simulink model "sm_car"  (R2025a)
settings: Solver=ode23t  StartTime=0.0  StopTime=400  MaxStep=0.4  RelTol=1e-3  AbsTol=1e-3  EnableMultiTasking=on
PreLoadFcn:
  | % Due to usability issue in Repeating Sequence block
  | warning('off','Simulink:Masking:Invalid');
  | 
  | % Eliminate unnecessary warnings in inactive variants
  | % Warnings generated only if you click through inactive variant
  | warning('off','MATLAB:nonExistentField');
  | warning('off','Simulink:Parameters:BlkParamUndefined');
PostLoadFcn:
  | set_param([bdroot '/Vehicle'],'popup_trailer','Off')
  | warning('off','sm:sli:setup:compile:LocalSolverNotSupported')
  | %sm_car_config_maneuver(bdroot,'WOT Braking');
  | sm_car_config_vehicle(bdroot,'false');
  | sm_car_config_logging(bdroot);
InitFcn:
  | sm_car_config_camera;
  | Vehicle = sm_car_vehcfg_checkConfig(Vehicle);
  | sm_car_check_tire_model(bdroot);
StartFcn:
  | tic;
StopFcn:
  | Elapsed_Sim_Time = toc;
  | % disp(['Elapsed Sim Time = ' num2str(Elapsed_Sim_Time)]);
undefined symbols (not defined in the file): Axle1D, AxleIn, Camera, Control, Driver, Free, Init, Maneuver, Pedal, RaceFix, RaceSpin, Scene, ShaftL1, ShaftL2, ShaftR1, ShaftR2, Soft, Stiff, Visual, X, xy_data_car_side, Y, Z
libraries: sm_lib x1546, nesl_utility x528, fl_lib x480, SimscapeFluids_lib x61, sdl_lib x49, simulink x29, ee_lib x7, simulink_extras x6, Linkage_Systems x4, Tire_1x2x x4, AntiRollBar_Systems x2, Linkage_Decoupled x2
(part 22 of 79)

== system sm_car/Vehicle/Vehicle/Chassis/Body/Body Geometry/CAD FSAE Achilles/Aero ==
  Aero Brackets : sm_lib/Body Elements/File Solid  ExtGeomFileName=FSAE_Aero_Brackets.STL  UnitType=Custom  ExtGeomFileUnits=m  StepReaderType=HEX  ExportConvexHullGeometry=off  InertiaType=PointMass  BasedOnType=Density  Density=700.769  DensityUnits=kg/m^3  Mass=0  MassUnits=kg  CenterOfMass=[0.988684, 1.00464/1.8, 2.92072]  CenterOfMassUnits=m  MomentsOfInertia=[478.463, 518.088, 108.52]  MomentsOfInertiaUnits=kg*m^2  ProductsOfInertia=[-18.6469, 0.0347848, 0.00267861]  ProductsOfInertiaUnits=kg*m^2  GraphicType=FromGeometry  MarkerShape=Sphere  MarkerSize=10  GraphicVisPropType=SimpleVisualProperties  GraphicDiffuseColor=[0.25 0.25 0.25]  GraphicOpacity=1  GraphicSpecularColor=[0.5 0.5 0.5 1.0]  GraphicAmbientColor=[0.15 0.15 0.15 1.0]  GraphicEmissiveColor=[0.0 0.0 0.0 1.0]  GraphicShininess=75  DoExposeReferenceFrame=on  SerializedFrames=<Frames/>
  Aero Surfaces : sm_lib/Body Elements/File Solid  ExtGeomFileName=FSAE_Aero_Surfaces.STL  UnitType=Custom  ExtGeomFileUnits=m  StepReaderType=HEX  ExportConvexHullGeometry=off  InertiaType=PointMass  BasedOnType=Density  Density=700.769  DensityUnits=kg/m^3  Mass=0  MassUnits=kg  CenterOfMass=[0.988684, 1.00464/1.8, 2.92072]  CenterOfMassUnits=m  MomentsOfInertia=[478.463, 518.088, 108.52]  MomentsOfInertiaUnits=kg*m^2  ProductsOfInertia=[-18.6469, 0.0347848, 0.00267861]  ProductsOfInertiaUnits=kg*m^2  GraphicType=FromGeometry  MarkerShape=Sphere  MarkerSize=10  GraphicVisPropType=SimpleVisualProperties  GraphicDiffuseColor=aero_clr  GraphicOpacity=aero_opc  GraphicSpecularColor=[0.5 0.5 0.5 1.0]  GraphicAmbientColor=[0.15 0.15 0.15 1.0]  GraphicEmissiveColor=[0.0 0.0 0.0 1.0]  GraphicShininess=75  DoExposeReferenceFrame=on  SerializedFrames=<Frames/>
  Ornament Left : sm_lib/Body Elements/Extruded Solid  ExtrusionType=General  PolygonNumSides=3  PolygonOuterRadius=1  PolygonOuterRadiusUnits=m  ExportEntireGeometry=off  ExtrusionCrossSection=extr_data_emblem_aero  ExtrusionCrossSectionUnits=m  ExportConvexHullGeometry=off  ExtrusionLength=0.005  ExtrusionLengthUnits=m  InertiaType=CalculateFromGeometry  BasedOnType=Density  Density=1000  DensityUnits=kg/m^3  Mass=1  MassUnits=kg  CenterOfMass=[0 0 0]  CenterOfMassUnits=m  MomentsOfInertia=[1 1 1]  MomentsOfInertiaUnits=kg*m^2  ProductsOfInertia=[0 0 0]  ProductsOfInertiaUnits=kg*m^2  GraphicType=FromGeometry  MarkerShape=Sphere  MarkerSize=10  GraphicVisPropType=SimpleVisualProperties  GraphicDiffuseColor=clr_emblem_aero  GraphicOpacity=opc_emblem_aero  GraphicSpecularColor=[0.5 0.5 0.5 1.0]  GraphicAmbientColor=[0.15 0.15 0.15 1.0]  GraphicEmissiveColor=[0.0 0.0 0.0 1.0]  GraphicShininess=75  DoExposeReferenceFrame=on  SerializedFrames=<Frames/>
  Ornament Right : sm_lib/Body Elements/Extruded Solid  ExtrusionType=General  PolygonNumSides=3  PolygonOuterRadius=1  PolygonOuterRadiusUnits=m  ExportEntireGeometry=off  ExtrusionCrossSection=extr_data_emblem_aero  ExtrusionCrossSectionUnits=m  ExportConvexHullGeometry=off  ExtrusionLength=0.005  ExtrusionLengthUnits=m  InertiaType=CalculateFromGeometry  BasedOnType=Density  Density=1000  DensityUnits=kg/m^3  Mass=1  MassUnits=kg  CenterOfMass=[0 0 0]  CenterOfMassUnits=m  MomentsOfInertia=[1 1 1]  MomentsOfInertiaUnits=kg*m^2  ProductsOfInertia=[0 0 0]  ProductsOfInertiaUnits=kg*m^2  GraphicType=FromGeometry  MarkerShape=Sphere  MarkerSize=10  GraphicVisPropType=SimpleVisualProperties  GraphicDiffuseColor=clr_emblem_aero  GraphicOpacity=opc_emblem_aero  GraphicSpecularColor=[0.5 0.5 0.5 1.0]  GraphicAmbientColor=[0.15 0.15 0.15 1.0]  GraphicEmissiveColor=[0.0 0.0 0.0 1.0]  GraphicShininess=75  DoExposeReferenceFrame=on  SerializedFrames=<Frames/>
  Transform Aero Ctr : sm_lib/Frames and Transforms/Rigid Transform  RotationMethod=None  FollAlignAxisA=+X  BaseAlignAxisA=+Y  FollAlignAxisB=+Y  BaseAlignAxisB=+Z  RotationStandardAxis=+X  RotationAngle=90  RotationAngleUnits=deg  RotationArbitraryAxis=[0 0 1]  RotationSequenceAxes=FollowerAxes  RotationSequence=XYX  RotationSequenceAngles=[0 0 0]  RotationSequenceAnglesUnits=deg  RotationMatrix=[1 0 0;0 1 0;0 0 1]  Quaternion=[1 0 0 0]  TranslationMethod=Cartesian  TranslationCartesianOffset=[-1.15 0 0.75]  TranslationCartesianOffsetUnits=m  TranslationStandardAxis=+Z  TranslationStandardOffset=0  TranslationStandardOffsetUnits=m  TranslationROffset=0  TranslationROffsetUnits=m  TranslationThetaOffset=0  TranslationThetaOffsetUnits=deg  TranslationZOffset=0  TranslationZOffsetUnits=m
  Transform Aero Left : sm_lib/Frames and Transforms/Rigid Transform  RotationMethod=RotationSequence  FollAlignAxisA=+X  BaseAlignAxisA=+Y  FollAlignAxisB=+Y  BaseAlignAxisB=+Z  RotationStandardAxis=+X  RotationAngle=90  RotationAngleUnits=deg  RotationArbitraryAxis=[0 0 1]  RotationSequenceAxes=FollowerAxes  RotationSequence=XYX  RotationSequenceAngles=[90 180 0]  RotationSequenceAnglesUnits=deg  RotationMatrix=[1 0 0;0 1 0;0 0 1]  Quaternion=[1 0 0 0]  TranslationMethod=Cartesian  TranslationCartesianOffset=[0 0.465 0]  TranslationCartesianOffsetUnits=m  TranslationStandardAxis=+Z  TranslationStandardOffset=0  TranslationStandardOffsetUnits=m  TranslationROffset=0  TranslationROffsetUnits=m  TranslationThetaOffset=0  TranslationThetaOffsetUnits=deg  TranslationZOffset=0  TranslationZOffsetUnits=m
  Transform Aero Right : sm_lib/Frames and Transforms/Rigid Transform  RotationMethod=StandardAxis  FollAlignAxisA=+X  BaseAlignAxisA=+Y  FollAlignAxisB=+Y  BaseAlignAxisB=+Z  RotationStandardAxis=+X  RotationAngle=90  RotationAngleUnits=deg  RotationArbitraryAxis=[0 0 1]  RotationSequenceAxes=FollowerAxes  RotationSequence=XYX  RotationSequenceAngles=[0 0 0]  RotationSequenceAnglesUnits=deg  RotationMatrix=[1 0 0;0 1 0;0 0 1]  Quaternion=[1 0 0 0]  TranslationMethod=Cartesian  TranslationCartesianOffset=[0 -0.465 0]  TranslationCartesianOffsetUnits=m  TranslationStandardAxis=+Z  TranslationStandardOffset=0  TranslationStandardOffsetUnits=m  TranslationROffset=0  TranslationROffsetUnits=m  TranslationThetaOffset=0  TranslationThetaOffsetUnits=deg  TranslationZOffset=0  TranslationZOffsetUnits=m
  R : PMIOPort  Side=Right
  connections:
  Ornament Right/RConn1 -- Transform Aero Right/RConn1
  Ornament Left/RConn1 -- Transform Aero Left/RConn1
  Aero Surfaces/RConn1 -- Transform Aero Ctr/LConn1 -- R/RConn1 -- Aero Brackets/RConn1
  Transform Aero Ctr/RConn1 -- Transform Aero Left/LConn1 -- Transform Aero Right/LConn1

== system sm_car/Vehicle/Vehicle/Chassis/Body/Body Geometry/CAD FSAE Achilles/Body ==
  Ornament Hood : sm_lib/Body Elements/Extruded Solid  ExtrusionType=General  PolygonNumSides=3  PolygonOuterRadius=1  PolygonOuterRadiusUnits=m  ExportEntireGeometry=off  ExtrusionCrossSection=extr_data_emblem_hood  ExtrusionCrossSectionUnits=m  ExportConvexHullGeometry=off  ExtrusionLength=0.01  ExtrusionLengthUnits=m  InertiaType=CalculateFromGeometry  BasedOnType=Density  Density=1000  DensityUnits=kg/m^3  Mass=1  MassUnits=kg  CenterOfMass=[0 0 0]  CenterOfMassUnits=m  MomentsOfInertia=[1 1 1]  MomentsOfInertiaUnits=kg*m^2  ProductsOfInertia=[0 0 0]  ProductsOfInertiaUnits=kg*m^2  GraphicType=FromGeometry  MarkerShape=Sphere  MarkerSize=10  GraphicVisPropType=SimpleVisualProperties  GraphicDiffuseColor=clr_emblem_hood  GraphicOpacity=opc_emblem_hood  GraphicSpecularColor=[0.5 0.5 0.5 1.0]  GraphicAmbientColor=[0.15 0.15 0.15 1.0]  GraphicEmissiveColor=[0.0 0.0 0.0 1.0]  GraphicShininess=75  DoExposeReferenceFrame=on  SerializedFrames=<Frames/>
  Shell : sm_lib/Body Elements/File Solid  ExtGeomFileName=FSAE_Body.STL  UnitType=Custom  ExtGeomFileUnits=m  StepReaderType=HEX  ExportConvexHullGeometry=off  InertiaType=PointMass  BasedOnType=Density  Density=700.769  DensityUnits=kg/m^3  Mass=0  MassUnits=kg  CenterOfMass=[0.988684, 1.00464/1.8, 2.92072]  CenterOfMassUnits=m  MomentsOfInertia=[478.463, 518.088, 108.52]  MomentsOfInertiaUnits=kg*m^2  ProductsOfInertia=[-18.6469, 0.0347848, 0.00267861]  ProductsOfInertiaUnits=kg*m^2  GraphicType=FromGeometry  MarkerShape=Sphere  MarkerSize=10  GraphicVisPropType=SimpleVisualProperties  GraphicDiffuseColor=[body_clr]  GraphicOpacity=body_opc  GraphicSpecularColor=[0.5 0.5 0.5 body_opc]  GraphicAmbientColor=[body_clr body_opc]  GraphicEmissiveColor=[0.0 0.0 0.0 body_opc]  GraphicShininess=50  DoExposeReferenceFrame=on  SerializedFrames=<Frames/>
  Transform Hood : sm_lib/Frames and Transforms/Rigid Transform  RotationMethod=RotationSequence  FollAlignAxisA=+X  BaseAlignAxisA=+Y  FollAlignAxisB=+Y  BaseAlignAxisB=+Z  RotationStandardAxis=+X  RotationAngle=90  RotationAngleUnits=deg  RotationArbitraryAxis=[0 0 1]  RotationSequenceAxes=FollowerAxes  RotationSequence=ZXY  RotationSequenceAngles=[90 9 0]  RotationSequenceAnglesUnits=deg  RotationMatrix=[1 0 0;0 1 0;0 0 1]  Quaternion=[1 0 0 0]  TranslationMethod=Cartesian  TranslationCartesianOffset=[0.75 0 0.56]  TranslationCartesianOffsetUnits=m  TranslationStandardAxis=+Z  TranslationStandardOffset=0  TranslationStandardOffsetUnits=m  TranslationROffset=0  TranslationROffsetUnits=m  TranslationThetaOffset=0  TranslationThetaOffsetUnits=deg  TranslationZOffset=0  TranslationZOffsetUnits=m
  R : PMIOPort  Side=Left
  connections:
  Shell/RConn1 -- R/RConn1 -- Transform Hood/LConn1
  Transform Hood/RConn1 -- Ornament Hood/RConn1

== system sm_car/Vehicle/Vehicle/Chassis/Body/Body Sensor/Roll Pitch/Calculate aPitch ==
  Roll Angle : Inport
  uvec : Inport  Port=2
  Asin : Trigonometry  Operator=asin
  Cos : Trigonometry  Operator=cos
  Divide : Product  Inputs=*/
  Divide1 : Product  Inputs=*/
  Selector : Selector  InputPortWidth=3  IndexOptions=Index vector (dialog)  Indices=[3]  OutputSizes=1
  magnitude : Fcn  Expr=sqrt(u(1)*u(1)+u(2)*u(2)+u(3)*u(3))
  Angle : Outport  VectorParamsAs1DForOutWhenUnconnected=off
  wires:
  Divide1/1 -> Asin/1
  uvec/1 -> magnitude/1, Selector/1
  magnitude/1 -> Divide1/2
  Selector/1 -> Divide/1
  Roll Angle/1 -> Cos/1
  Asin/1 -> Angle/1
  Divide/1 -> Divide1/1
  Cos/1 -> Divide/2

== system sm_car/Vehicle/Vehicle/Chassis/Body/Body Sensor/Roll Pitch/Calculate aRoll ==
  uvec : Inport
  Demux : Demux  Outputs=3
  Mux : Mux  Inputs=2
  Trigonometric Function1 : Trigonometry  Operator=atan2
  magnitude : Fcn  Expr=sqrt(u(1)*u(1)+u(2)*u(2))
  Angle : Outport  VectorParamsAs1DForOutWhenUnconnected=off
  wires:
  Demux/2 -> Mux/2
  magnitude/1 -> Trigonometric Function1/2
  Mux/1 -> magnitude/1
  Demux/3 -> Trigonometric Function1/1
  Trigonometric Function1/1 -> Angle/1
  uvec/1 -> Demux/1
  Demux/1 -> Mux/1

== system sm_car/Vehicle/Vehicle/Chassis/Body/Passenger FL/None/Body Sensor Empty ==
  Constant{,1..14} (15 alike) : Constant  Value=0
  Reference Frame : sm_lib/Frames and Transforms/Reference Frame
  Signal Specification : SignalSpecification  Unit=rad
  Signal Specification1 : SignalSpecification  Unit=rad
  Signal Specification2 : SignalSpecification  Unit=rad
  Signal Specification3 : SignalSpecification  Unit=rad/s
  Signal Specification4 : SignalSpecification  Unit=rad/s
  Signal Specification5 : SignalSpecification  Unit=rad/s
  B : PMIOPort  Side=Left
  Bus Element Out : Outport  VectorParamsAs1DForOutWhenUnconnected=off  PortName=Body  Element=x
  Bus Element Out1 : Outport  VectorParamsAs1DForOutWhenUnconnected=off  PortName=Body  Element=y
  Bus Element Out2 : Outport  VectorParamsAs1DForOutWhenUnconnected=off  PortName=Body  Element=z
  Bus Element Out3 : Outport  VectorParamsAs1DForOutWhenUnconnected=off  PortName=Body  Element=vx
  Bus Element Out4 : Outport  VectorParamsAs1DForOutWhenUnconnected=off  PortName=Body  Element=vy
  Bus Element Out5 : Outport  VectorParamsAs1DForOutWhenUnconnected=off  PortName=Body  Element=vz
  Bus Element Out6 : Outport  VectorParamsAs1DForOutWhenUnconnected=off  PortName=Body  Element=gx
  Bus Element Out7 : Outport  VectorParamsAs1DForOutWhenUnconnected=off  PortName=Body  Element=gy
  Bus Element Out8 : Outport  VectorParamsAs1DForOutWhenUnconnected=off  PortName=Body  Element=gz
  Bus Element Out9 : Outport  VectorParamsAs1DForOutWhenUnconnected=off  PortName=Body  Element=nRoll
  Bus Element Out10 : Outport  VectorParamsAs1DForOutWhenUnconnected=off  PortName=Body  Element=nPitch
  Bus Element Out11 : Outport  VectorParamsAs1DForOutWhenUnconnected=off  PortName=Body  Element=nYaw
  Bus Element Out12 : Outport  VectorParamsAs1DForOutWhenUnconnected=off  PortName=Body  Element=aRoll
  Bus Element Out13 : Outport  VectorParamsAs1DForOutWhenUnconnected=off  PortName=Body  Element=aPitch
  Bus Element Out14 : Outport  VectorParamsAs1DForOutWhenUnconnected=off  PortName=Body  Element=aYaw
  wires:
  Constant2/1 -> Signal Specification/1
  Constant3/1 -> Signal Specification1/1
  Constant5/1 -> Signal Specification4/1
  Constant4/1 -> Signal Specification3/1
  Constant1/1 -> Signal Specification5/1
  Constant/1 -> Signal Specification2/1
  Signal Specification5/1 -> Bus Element Out11/1
  Signal Specification4/1 -> Bus Element Out10/1
  Signal Specification3/1 -> Bus Element Out9/1
  Signal Specification2/1 -> Bus Element Out14/1
  Signal Specification1/1 -> Bus Element Out13/1
  Signal Specification/1 -> Bus Element Out12/1
  Constant9/1 -> Bus Element Out3/1
  Constant6/1 -> Bus Element Out/1
  Constant8/1 -> Bus Element Out2/1
  Constant10/1 -> Bus Element Out4/1
  Constant13/1 -> Bus Element Out7/1
  Constant7/1 -> Bus Element Out1/1
  Constant12/1 -> Bus Element Out6/1
  Constant11/1 -> Bus Element Out5/1
  Constant14/1 -> Bus Element Out8/1
  connections:
  B/RConn1 -- Reference Frame/RConn1

== system sm_car/Vehicle/Vehicle/Chassis/Body/Passenger FR/None/Body Sensor Empty ==
  Constant{,1..14} (15 alike) : Constant  Value=0
  Reference Frame : sm_lib/Frames and Transforms/Reference Frame
  Signal Specification : SignalSpecification  Unit=rad
  Signal Specification1 : SignalSpecification  Unit=rad
  Signal Specification2 : SignalSpecification  Unit=rad
  Signal Specification3 : SignalSpecification  Unit=rad/s
  Signal Specification4 : SignalSpecification  Unit=rad/s
  Signal Specification5 : SignalSpecification  Unit=rad/s
  B : PMIOPort  Side=Left
  Bus Element Out : Outport  VectorParamsAs1DForOutWhenUnconnected=off  PortName=Body  Element=x
  Bus Element Out1 : Outport  VectorParamsAs1DForOutWhenUnconnected=off  PortName=Body  Element=y
  Bus Element Out2 : Outport  VectorParamsAs1DForOutWhenUnconnected=off  PortName=Body  Element=z
  Bus Element Out3 : Outport  VectorParamsAs1DForOutWhenUnconnected=off  PortName=Body  Element=vx
  Bus Element Out4 : Outport  VectorParamsAs1DForOutWhenUnconnected=off  PortName=Body  Element=vy
  Bus Element Out5 : Outport  VectorParamsAs1DForOutWhenUnconnected=off  PortName=Body  Element=vz
  Bus Element Out6 : Outport  VectorParamsAs1DForOutWhenUnconnected=off  PortName=Body  Element=gx
  Bus Element Out7 : Outport  VectorParamsAs1DForOutWhenUnconnected=off  PortName=Body  Element=gy
  Bus Element Out8 : Outport  VectorParamsAs1DForOutWhenUnconnected=off  PortName=Body  Element=gz
  Bus Element Out9 : Outport  VectorParamsAs1DForOutWhenUnconnected=off  PortName=Body  Element=nRoll
  Bus Element Out10 : Outport  VectorParamsAs1DForOutWhenUnconnected=off  PortName=Body  Element=nPitch
  Bus Element Out11 : Outport  VectorParamsAs1DForOutWhenUnconnected=off  PortName=Body  Element=nYaw
  Bus Element Out12 : Outport  VectorParamsAs1DForOutWhenUnconnected=off  PortName=Body  Element=aRoll
  Bus Element Out13 : Outport  VectorParamsAs1DForOutWhenUnconnected=off  PortName=Body  Element=aPitch
  Bus Element Out14 : Outport  VectorParamsAs1DForOutWhenUnconnected=off  PortName=Body  Element=aYaw
  wires:
  Constant2/1 -> Signal Specification/1
  Constant3/1 -> Signal Specification1/1
  Constant5/1 -> Signal Specification4/1
  Constant4/1 -> Signal Specification3/1
  Constant1/1 -> Signal Specification5/1
  Constant/1 -> Signal Specification2/1
  Signal Specification5/1 -> Bus Element Out11/1
  Signal Specification4/1 -> Bus Element Out10/1
  Signal Specification3/1 -> Bus Element Out9/1
  Signal Specification2/1 -> Bus Element Out14/1
  Signal Specification1/1 -> Bus Element Out13/1
  Signal Specification/1 -> Bus Element Out12/1
  Constant9/1 -> Bus Element Out3/1
  Constant6/1 -> Bus Element Out/1
  Constant8/1 -> Bus Element Out2/1
  Constant10/1 -> Bus Element Out4/1
  Constant13/1 -> Bus Element Out7/1
  Constant7/1 -> Bus Element Out1/1
  Constant12/1 -> Bus Element Out6/1
  Constant11/1 -> Bus Element Out5/1
  Constant14/1 -> Bus Element Out8/1
  connections:
  B/RConn1 -- Reference Frame/RConn1

== system sm_car/Vehicle/Vehicle/Chassis/Body/Passenger RL/None/Body Sensor Empty ==
  Constant{,1..14} (15 alike) : Constant  Value=0
  Reference Frame : sm_lib/Frames and Transforms/Reference Frame
  Signal Specification : SignalSpecification  Unit=rad
  Signal Specification1 : SignalSpecification  Unit=rad
  Signal Specification2 : SignalSpecification  Unit=rad
  Signal Specification3 : SignalSpecification  Unit=rad/s
  Signal Specification4 : SignalSpecification  Unit=rad/s
  Signal Specification5 : SignalSpecification  Unit=rad/s
  B : PMIOPort  Side=Left
  Bus Element Out : Outport  VectorParamsAs1DForOutWhenUnconnected=off  PortName=Body  Element=x
  Bus Element Out1 : Outport  VectorParamsAs1DForOutWhenUnconnected=off  PortName=Body  Element=y
  Bus Element Out2 : Outport  VectorParamsAs1DForOutWhenUnconnected=off  PortName=Body  Element=z
  Bus Element Out3 : Outport  VectorParamsAs1DForOutWhenUnconnected=off  PortName=Body  Element=vx
  Bus Element Out4 : Outport  VectorParamsAs1DForOutWhenUnconnected=off  PortName=Body  Element=vy
  Bus Element Out5 : Outport  VectorParamsAs1DForOutWhenUnconnected=off  PortName=Body  Element=vz
  Bus Element Out6 : Outport  VectorParamsAs1DForOutWhenUnconnected=off  PortName=Body  Element=gx
  Bus Element Out7 : Outport  VectorParamsAs1DForOutWhenUnconnected=off  PortName=Body  Element=gy
  Bus Element Out8 : Outport  VectorParamsAs1DForOutWhenUnconnected=off  PortName=Body  Element=gz
  Bus Element Out9 : Outport  VectorParamsAs1DForOutWhenUnconnected=off  PortName=Body  Element=nRoll
  Bus Element Out10 : Outport  VectorParamsAs1DForOutWhenUnconnected=off  PortName=Body  Element=nPitch
  Bus Element Out11 : Outport  VectorParamsAs1DForOutWhenUnconnected=off  PortName=Body  Element=nYaw
  Bus Element Out12 : Outport  VectorParamsAs1DForOutWhenUnconnected=off  PortName=Body  Element=aRoll
  Bus Element Out13 : Outport  VectorParamsAs1DForOutWhenUnconnected=off  PortName=Body  Element=aPitch
  Bus Element Out14 : Outport  VectorParamsAs1DForOutWhenUnconnected=off  PortName=Body  Element=aYaw
  wires:
  Constant2/1 -> Signal Specification/1
  Constant3/1 -> Signal Specification1/1
  Constant5/1 -> Signal Specification4/1
  Constant4/1 -> Signal Specification3/1
  Constant1/1 -> Signal Specification5/1
  Constant/1 -> Signal Specification2/1
  Signal Specification5/1 -> Bus Element Out11/1
  Signal Specification4/1 -> Bus Element Out10/1
  Signal Specification3/1 -> Bus Element Out9/1
  Signal Specification2/1 -> Bus Element Out14/1
  Signal Specification1/1 -> Bus Element Out13/1
  Signal Specification/1 -> Bus Element Out12/1
  Constant9/1 -> Bus Element Out3/1
  Constant6/1 -> Bus Element Out/1
  Constant8/1 -> Bus Element Out2/1
  Constant10/1 -> Bus Element Out4/1
  Constant13/1 -> Bus Element Out7/1
  Constant7/1 -> Bus Element Out1/1
  Constant12/1 -> Bus Element Out6/1
  Constant11/1 -> Bus Element Out5/1
  Constant14/1 -> Bus Element Out8/1
  connections:
  B/RConn1 -- Reference Frame/RConn1

== system sm_car/Vehicle/Vehicle/Chassis/Body/Passenger RR/None/Body Sensor Empty ==
  Constant{,1..14} (15 alike) : Constant  Value=0
  Reference Frame : sm_lib/Frames and Transforms/Reference Frame
  Signal Specification : SignalSpecification  Unit=rad
  Signal Specification1 : SignalSpecification  Unit=rad
  Signal Specification2 : SignalSpecification  Unit=rad
  Signal Specification3 : SignalSpecification  Unit=rad/s
  Signal Specification4 : SignalSpecification  Unit=rad/s
  Signal Specification5 : SignalSpecification  Unit=rad/s
  B : PMIOPort  Side=Left
  Bus Element Out : Outport  VectorParamsAs1DForOutWhenUnconnected=off  PortName=Body  Element=x
  Bus Element Out1 : Outport  VectorParamsAs1DForOutWhenUnconnected=off  PortName=Body  Element=y
  Bus Element Out2 : Outport  VectorParamsAs1DForOutWhenUnconnected=off  PortName=Body  Element=z
  Bus Element Out3 : Outport  VectorParamsAs1DForOutWhenUnconnected=off  PortName=Body  Element=vx
  Bus Element Out4 : Outport  VectorParamsAs1DForOutWhenUnconnected=off  PortName=Body  Element=vy
  Bus Element Out5 : Outport  VectorParamsAs1DForOutWhenUnconnected=off  PortName=Body  Element=vz
  Bus Element Out6 : Outport  VectorParamsAs1DForOutWhenUnconnected=off  PortName=Body  Element=gx
  Bus Element Out7 : Outport  VectorParamsAs1DForOutWhenUnconnected=off  PortName=Body  Element=gy
  Bus Element Out8 : Outport  VectorParamsAs1DForOutWhenUnconnected=off  PortName=Body  Element=gz
  Bus Element Out9 : Outport  VectorParamsAs1DForOutWhenUnconnected=off  PortName=Body  Element=nRoll
  Bus Element Out10 : Outport  VectorParamsAs1DForOutWhenUnconnected=off  PortName=Body  Element=nPitch
  Bus Element Out11 : Outport  VectorParamsAs1DForOutWhenUnconnected=off  PortName=Body  Element=nYaw
  Bus Element Out12 : Outport  VectorParamsAs1DForOutWhenUnconnected=off  PortName=Body  Element=aRoll
  Bus Element Out13 : Outport  VectorParamsAs1DForOutWhenUnconnected=off  PortName=Body  Element=aPitch
  Bus Element Out14 : Outport  VectorParamsAs1DForOutWhenUnconnected=off  PortName=Body  Element=aYaw
  wires:
  Constant2/1 -> Signal Specification/1
  Constant3/1 -> Signal Specification1/1
  Constant5/1 -> Signal Specification4/1
  Constant4/1 -> Signal Specification3/1
  Constant1/1 -> Signal Specification5/1
  Constant/1 -> Signal Specification2/1
  Signal Specification5/1 -> Bus Element Out11/1
  Signal Specification4/1 -> Bus Element Out10/1
  Signal Specification3/1 -> Bus Element Out9/1
  Signal Specification2/1 -> Bus Element Out14/1
  Signal Specification1/1 -> Bus Element Out13/1
  Signal Specification/1 -> Bus Element Out12/1
  Constant9/1 -> Bus Element Out3/1
  Constant6/1 -> Bus Element Out/1
  Constant8/1 -> Bus Element Out2/1
  Constant10/1 -> Bus Element Out4/1
  Constant13/1 -> Bus Element Out7/1
  Constant7/1 -> Bus Element Out1/1
  Constant12/1 -> Bus Element Out6/1
  Constant11/1 -> Bus Element Out5/1
  Constant14/1 -> Bus Element Out8/1
  connections:
  B/RConn1 -- Reference Frame/RConn1

== system sm_car/Vehicle/Vehicle/Chassis/Damper/Decoupled/Damper A1 Heave/Force Endstop NL ==
  note: Sensing
  Ctrl : Inport
  Bumpstop : sdl_lib/Couplings & Drives/Springs & Dampers/Nonlinear Translational Spring  parameterization=sdl.enum.polynomialTLU.tlu  symmetry=sdl.enum.symmetry.twoSided  coefficient_vector=[100, 0, 10, 0, 1] N/m  tension_coefficient_vector=[100, 0, 10, 0, 1] N/m  compression_coefficient_vector=[1000, -10, 100, 0, 0] N/m  deformation_vector=xEndstop m  force_vector=fEndstop N  interp_method=simscape.enum.interpolation.linear  extrap_method=simscape.enum.extrapolation.linear  x_specify=on  x_priority=None  x=0 m  x_nominal_specify=off  x_nominal_value=1  x_nominal_unit=m
      settings: InternalSimscapePortConfiguration="{\"Bottom\":[],\"Left\":[{\"id\":\"R\",\"label\":\"R\",\"type\":\"foundation.mechanical.translational.translational\"}],\"Right\":[{\"id\":\"C\",\"label\":\"C\",\"type\":\"foundation.mechanical.translational.translational\"}],\"Top\":[]}"
  Force Source : fl_lib/Mechanical/Mechanical Sources/Ideal Force Source
  Force Bumpstop : fl_lib/Mechanical/Mechanical Sensors/Ideal Force Sensor
  Force Damper : fl_lib/Mechanical/Mechanical Sensors/Ideal Force Sensor
  Motion Damper : fl_lib/Mechanical/Mechanical Sensors/Ideal Translational Motion Sensor  reference=foundation.enum.MeasurementReference.difference  acceleration_port=false  velocity_port=true  position_port=true  offset=dam_x0 m
  PS-Simulink Converter : nesl_utility/PS-Simulink Converter  PhysicalDomain=network_engine_domain  SubClassName=ps_output  LeftPortType=input  RightPortType=output  PseudoPeriodic=off  Frequencies=[]  VectorFormat=1-D array  Unit=N  AffineConversion=off
  PS-Simulink Converter1 : nesl_utility/PS-Simulink Converter  PhysicalDomain=network_engine_domain  SubClassName=ps_output  LeftPortType=input  RightPortType=output  PseudoPeriodic=off  Frequencies=[]  VectorFormat=1-D array  Unit=N  AffineConversion=off
  PS-Simulink Converter2 : nesl_utility/PS-Simulink Converter  PhysicalDomain=network_engine_domain  SubClassName=ps_output  LeftPortType=input  RightPortType=output  PseudoPeriodic=off  Frequencies=[]  VectorFormat=1-D array  Unit=m/s  AffineConversion=off
  PS-Simulink Converter3 : nesl_utility/PS-Simulink Converter  PhysicalDomain=network_engine_domain  SubClassName=ps_output  LeftPortType=input  RightPortType=output  PseudoPeriodic=off  Frequencies=[]  VectorFormat=1-D array  Unit=m  AffineConversion=off
  Simulink-PS Converter : nesl_utility/Simulink-PS Converter  PhysicalDomain=network_engine_domain  SubClassName=ps_input  LeftPortType=input  RightPortType=output  PseudoPeriodic=off  Frequencies=[]  NoiseDistribution=none  NoiseParameters=[]  Unit=N  AffineConversion=off  FilteringAndDerivatives=filter  SimscapeFilterOrder=1  InputFilterTimeConstant=0.01  UdotUserProvided=0
  R : PMIOPort  Side=Left
  C : PMIOPort  Port=2  Side=Right
  Out Bus Element : Outport  VectorParamsAs1DForOutWhenUnconnected=off  PortName=meas  Element=FDamper
  Out Bus Element1 : Outport  VectorParamsAs1DForOutWhenUnconnected=off  PortName=meas  Element=FBumpstop
  Out Bus Element2 : Outport  VectorParamsAs1DForOutWhenUnconnected=off  PortName=meas  Element=xDamper
  Out Bus Element3 : Outport  VectorParamsAs1DForOutWhenUnconnected=off  PortName=meas  Element=vDamper
  wires:
  PS-Simulink Converter1/1 -> Out Bus Element1/1
  PS-Simulink Converter3/1 -> Out Bus Element2/1
  PS-Simulink Converter2/1 -> Out Bus Element3/1
  PS-Simulink Converter/1 -> Out Bus Element/1
  Ctrl/1 -> Simulink-PS Converter/1
  connections:
  Simulink-PS Converter/RConn1 -- Force Source/RConn1
  Force Source/RConn2 -- Bumpstop/LConn1 -- R/RConn1 -- Motion Damper/LConn1
  Force Source/LConn1 -- Force Damper/RConn1
  Bumpstop/RConn1 -- Force Bumpstop/RConn1
  PS-Simulink Converter/LConn1 -- Force Damper/RConn2
  PS-Simulink Converter3/LConn1 -- Motion Damper/RConn3
  PS-Simulink Converter1/LConn1 -- Force Bumpstop/RConn2
  PS-Simulink Converter2/LConn1 -- Motion Damper/RConn2
  Force Damper/LConn1 -- C/RConn1 -- Force Bumpstop/LConn1 -- Motion Damper/RConn1

== system sm_car/Vehicle/Vehicle/Chassis/Damper/Decoupled/Damper A1 Heave/Linear ==
  note: Sensing
  Ctrl : Inport
  Bumpstop : fl_lib/Mechanical/Translational Elements/Translational Hard Stop  upper_bnd=bs_lim_upper m  lower_bnd=bs_lim_lower m  model=1  stiff_up=bs_k_upper N/m  stiff_low=bs_k_lower N/m  D_up=bs_b_upper N/(m/s)  D_low=bs_b_lower N/(m/s)  transition=bs_region m  coeff_rest=0.7  v_tol=0.001 m/s  f_tol=0.001 N  v_specify=off  v_priority=None  v=0 m/s  v_nominal_specify=off  v_nominal_value=1  v_nominal_unit=m/s  f_specify=off  f_priority=None  f=0 N  f_nominal_specify=off  f_nominal_value=1  f_nominal_unit=N  x_specify=off  x_priority=High  x=0 m  x_nominal_specify=off  x_nominal_value=1  x_nominal_unit=m  M_specify=off  M_priority=None  M=0
  Damper : fl_lib/Mechanical/Translational Elements/Translational Damper  D=dam_b N/(m/s)  v_specify=off  v_priority=None  v=0 m/s  v_nominal_specify=off  v_nominal_value=1  v_nominal_unit=m/s  f_specify=off  f_priority=None  f=0 N  f_nominal_specify=off  f_nominal_value=1  f_nominal_unit=N
  Force Bumpstop : fl_lib/Mechanical/Mechanical Sensors/Ideal Force Sensor
  Force Damper : fl_lib/Mechanical/Mechanical Sensors/Ideal Force Sensor
  Motion Damper : fl_lib/Mechanical/Mechanical Sensors/Ideal Translational Motion Sensor  reference=foundation.enum.MeasurementReference.difference  acceleration_port=false  velocity_port=true  position_port=true  offset=dam_x0 m
  PS-Simulink Converter : nesl_utility/PS-Simulink Converter  PhysicalDomain=network_engine_domain  SubClassName=ps_output  LeftPortType=input  RightPortType=output  PseudoPeriodic=off  Frequencies=[]  VectorFormat=1-D array  Unit=N  AffineConversion=off
  PS-Simulink Converter1 : nesl_utility/PS-Simulink Converter  PhysicalDomain=network_engine_domain  SubClassName=ps_output  LeftPortType=input  RightPortType=output  PseudoPeriodic=off  Frequencies=[]  VectorFormat=1-D array  Unit=N  AffineConversion=off
  PS-Simulink Converter2 : nesl_utility/PS-Simulink Converter  PhysicalDomain=network_engine_domain  SubClassName=ps_output  LeftPortType=input  RightPortType=output  PseudoPeriodic=off  Frequencies=[]  VectorFormat=1-D array  Unit=m/s  AffineConversion=off
  PS-Simulink Converter3 : nesl_utility/PS-Simulink Converter  PhysicalDomain=network_engine_domain  SubClassName=ps_output  LeftPortType=input  RightPortType=output  PseudoPeriodic=off  Frequencies=[]  VectorFormat=1-D array  Unit=m  AffineConversion=off
  Terminator : Terminator
  R : PMIOPort  Side=Left
  C : PMIOPort  Port=2  Side=Right
  Out Bus Element : Outport  VectorParamsAs1DForOutWhenUnconnected=off  PortName=meas  Element=FDamper
  Out Bus Element1 : Outport  VectorParamsAs1DForOutWhenUnconnected=off  PortName=meas  Element=FBumpstop
  Out Bus Element2 : Outport  VectorParamsAs1DForOutWhenUnconnected=off  PortName=meas  Element=xDamper
  Out Bus Element3 : Outport  VectorParamsAs1DForOutWhenUnconnected=off  PortName=meas  Element=vDamper
  wires:
  PS-Simulink Converter1/1 -> Out Bus Element1/1
  PS-Simulink Converter3/1 -> Out Bus Element2/1
  PS-Simulink Converter2/1 -> Out Bus Element3/1
  PS-Simulink Converter/1 -> Out Bus Element/1
  Ctrl/1 -> Terminator/1
  connections:
  R/RConn1 -- Motion Damper/LConn1 -- Bumpstop/LConn1 -- Damper/LConn1
  Force Damper/RConn1 -- Damper/RConn1
  Force Bumpstop/RConn1 -- Bumpstop/RConn1
  PS-Simulink Converter/LConn1 -- Force Damper/RConn2
  PS-Simulink Converter3/LConn1 -- Motion Damper/RConn3
  PS-Simulink Converter1/LConn1 -- Force Bumpstop/RConn2
  PS-Simulink Converter2/LConn1 -- Motion Damper/RConn2
  Force Damper/LConn1 -- C/RConn1 -- Force Bumpstop/LConn1 -- Motion Damper/RConn1

== system sm_car/Vehicle/Vehicle/Chassis/Damper/Decoupled/Damper A1 Heave/None ==
  note: Sensor inserted simply to ensure
      | all blocks are connected to a network
  Ctrl : Inport
  Constant{1..4} (4 alike) : Constant  Value=0
  Ideal Translational Motion Sensor : fl_lib/Mechanical/Mechanical Sensors/Ideal Translational Motion Sensor  reference=foundation.enum.MeasurementReference.difference  acceleration_port=false  velocity_port=true  position_port=true  offset=0 m
  PS-Simulink Converter2 : nesl_utility/PS-Simulink Converter  PhysicalDomain=network_engine_domain  SubClassName=ps_output  LeftPortType=input  RightPortType=output  PseudoPeriodic=off  Frequencies=[]  VectorFormat=1-D array  Unit=1  AffineConversion=off
  PS-Simulink Converter3 : nesl_utility/PS-Simulink Converter  PhysicalDomain=network_engine_domain  SubClassName=ps_output  LeftPortType=input  RightPortType=output  PseudoPeriodic=off  Frequencies=[]  VectorFormat=1-D array  Unit=1  AffineConversion=off
  Terminator : Terminator
  Terminator1 : Terminator
  Terminator2 : Terminator
  R : PMIOPort  Side=Left
  C : PMIOPort  Port=2  Side=Right
  Out Bus Element : Outport  VectorParamsAs1DForOutWhenUnconnected=off  PortName=meas  Element=FDamper
  Out Bus Element1 : Outport  VectorParamsAs1DForOutWhenUnconnected=off  PortName=meas  Element=FBumpstop
  Out Bus Element2 : Outport  VectorParamsAs1DForOutWhenUnconnected=off  PortName=meas  Element=xDamper
  Out Bus Element3 : Outport  VectorParamsAs1DForOutWhenUnconnected=off  PortName=meas  Element=vDamper
  wires:
  PS-Simulink Converter2/1 -> Terminator1/1
  PS-Simulink Converter3/1 -> Terminator2/1
  Constant2/1 -> Out Bus Element1/1
  Constant4/1 -> Out Bus Element2/1
  Constant3/1 -> Out Bus Element3/1
  Constant1/1 -> Out Bus Element/1
  Ctrl/1 -> Terminator/1
  connections:
  C/RConn1 -- Ideal Translational Motion Sensor/RConn1
  R/RConn1 -- Ideal Translational Motion Sensor/LConn1
  PS-Simulink Converter3/LConn1 -- Ideal Translational Motion Sensor/RConn3
  Ideal Translational Motion Sensor/RConn2 -- PS-Simulink Converter2/LConn1

== system sm_car/Vehicle/Vehicle/Chassis/Damper/Decoupled/Damper A1 Heave/Nonlinear ==
  note: Sensing
  Ctrl : Inport
  Bumpstop : fl_lib/Mechanical/Translational Elements/Translational Hard Stop  upper_bnd=bs_lim_upper m  lower_bnd=bs_lim_lower m  model=1  stiff_up=bs_k_upper N/m  stiff_low=bs_k_lower N/m  D_up=bs_b_upper N/(m/s)  D_low=bs_b_lower N/(m/s)  transition=bs_region m  coeff_rest=0.7  v_tol=0.001 m/s  f_tol=0.001 N  v_specify=off  v_priority=None  v=0 m/s  v_nominal_specify=off  v_nominal_value=1  v_nominal_unit=m/s  f_specify=off  f_priority=None  f=0 N  f_nominal_specify=off  f_nominal_value=1  f_nominal_unit=N  x_specify=off  x_priority=High  x=0 m  x_nominal_specify=off  x_nominal_value=1  x_nominal_unit=m  M_specify=off  M_priority=None  M=0
  Damper : sdl_lib/Couplings & Drives/Springs & Dampers/Nonlinear Translational Damper  parameterization=2  symmetry=1  coefficient_vector=[10, 0, 1, 0, .1] N/(m/s)  extension_coefficient_vector=[10, 0, 1, 0, .1] N/(m/s)  contraction_coefficient_vector=[100, -1, 10, 0, 0] N/(m/s)  velocity_vector=velocity_vector m/s  force_vector=force_vector N  interp_method=simscape.enum.interpolation.linear  extrap_method=simscape.enum.extrapolation.linear
      settings: InternalSimscapePortConfiguration="{\"Bottom\":[],\"Left\":[{\"id\":\"R\",\"label\":\"R\",\"type\":\"foundation.mechanical.translational.translational\"}],\"Right\":[{\"id\":\"C\",\"label\":\"C\",\"type\":\"foundation.mechanical.translational.translational\"}],\"Top\":[]}"
  Force Bumpstop : fl_lib/Mechanical/Mechanical Sensors/Ideal Force Sensor
  Force Damper : fl_lib/Mechanical/Mechanical Sensors/Ideal Force Sensor
  Motion Damper : fl_lib/Mechanical/Mechanical Sensors/Ideal Translational Motion Sensor  reference=foundation.enum.MeasurementReference.difference  acceleration_port=false  velocity_port=true  position_port=true  offset=dam_x0 m
  PS-Simulink Converter : nesl_utility/PS-Simulink Converter  PhysicalDomain=network_engine_domain  SubClassName=ps_output  LeftPortType=input  RightPortType=output  PseudoPeriodic=off  Frequencies=[]  VectorFormat=1-D array  Unit=N  AffineConversion=off
  PS-Simulink Converter1 : nesl_utility/PS-Simulink Converter  PhysicalDomain=network_engine_domain  SubClassName=ps_output  LeftPortType=input  RightPortType=output  PseudoPeriodic=off  Frequencies=[]  VectorFormat=1-D array  Unit=N  AffineConversion=off
  PS-Simulink Converter2 : nesl_utility/PS-Simulink Converter  PhysicalDomain=network_engine_domain  SubClassName=ps_output  LeftPortType=input  RightPortType=output  PseudoPeriodic=off  Frequencies=[]  VectorFormat=1-D array  Unit=m/s  AffineConversion=off
  PS-Simulink Converter3 : nesl_utility/PS-Simulink Converter  PhysicalDomain=network_engine_domain  SubClassName=ps_output  LeftPortType=input  RightPortType=output  PseudoPeriodic=off  Frequencies=[]  VectorFormat=1-D array  Unit=m  AffineConversion=off
  Terminator : Terminator
  R : PMIOPort  Side=Left
  C : PMIOPort  Port=2  Side=Right
  Out Bus Element : Outport  VectorParamsAs1DForOutWhenUnconnected=off  PortName=meas  Element=FDamper
  Out Bus Element1 : Outport  VectorParamsAs1DForOutWhenUnconnected=off  PortName=meas  Element=FBumpstop
  Out Bus Element2 : Outport  VectorParamsAs1DForOutWhenUnconnected=off  PortName=meas  Element=xDamper
  Out Bus Element3 : Outport  VectorParamsAs1DForOutWhenUnconnected=off  PortName=meas  Element=vDamper
  wires:
  Ctrl/1 -> Terminator/1
  PS-Simulink Converter/1 -> Out Bus Element/1
  PS-Simulink Converter2/1 -> Out Bus Element3/1
  PS-Simulink Converter3/1 -> Out Bus Element2/1
  PS-Simulink Converter1/1 -> Out Bus Element1/1
  connections:
  Motion Damper/RConn1 -- Force Bumpstop/LConn1 -- C/RConn1 -- Force Damper/LConn1
  PS-Simulink Converter2/LConn1 -- Motion Damper/RConn2
  PS-Simulink Converter1/LConn1 -- Force Bumpstop/RConn2
  PS-Simulink Converter3/LConn1 -- Motion Damper/RConn3
  PS-Simulink Converter/LConn1 -- Force Damper/RConn2
  Force Bumpstop/RConn1 -- Bumpstop/RConn1
  Damper/RConn1 -- Force Damper/RConn1
  Bumpstop/LConn1 -- Motion Damper/LConn1 -- R/RConn1 -- Damper/LConn1

== system sm_car/Vehicle/Vehicle/Chassis/Damper/Decoupled/Damper A1 Heave/Nonlinear Endstop NL ==
  note: Sensing
  Ctrl : Inport
  Bumpstop : sdl_lib/Couplings & Drives/Springs & Dampers/Nonlinear Translational Spring  parameterization=sdl.enum.polynomialTLU.tlu  symmetry=sdl.enum.symmetry.twoSided  coefficient_vector=[100, 0, 10, 0, 1] N/m  tension_coefficient_vector=[100, 0, 10, 0, 1] N/m  compression_coefficient_vector=[1000, -10, 100, 0, 0] N/m  deformation_vector=xEndstop m  force_vector=fEndstop N  interp_method=simscape.enum.interpolation.linear  extrap_method=simscape.enum.extrapolation.linear  x_specify=on  x_priority=None  x=0 m  x_nominal_specify=off  x_nominal_value=1  x_nominal_unit=m
      settings: InternalSimscapePortConfiguration="{\"Bottom\":[],\"Left\":[{\"id\":\"R\",\"label\":\"R\",\"type\":\"foundation.mechanical.translational.translational\"}],\"Right\":[{\"id\":\"C\",\"label\":\"C\",\"type\":\"foundation.mechanical.translational.translational\"}],\"Top\":[]}"
  Damper : sdl_lib/Couplings & Drives/Springs & Dampers/Nonlinear Translational Damper  parameterization=2  symmetry=1  coefficient_vector=[10, 0, 1, 0, .1] N/(m/s)  extension_coefficient_vector=[10, 0, 1, 0, .1] N/(m/s)  contraction_coefficient_vector=[100, -1, 10, 0, 0] N/(m/s)  velocity_vector=velocity_vector m/s  force_vector=force_vector N  interp_method=simscape.enum.interpolation.linear  extrap_method=simscape.enum.extrapolation.linear
      settings: InternalSimscapePortConfiguration="{\"Bottom\":[],\"Left\":[{\"id\":\"R\",\"label\":\"R\",\"type\":\"foundation.mechanical.translational.translational\"}],\"Right\":[{\"id\":\"C\",\"label\":\"C\",\"type\":\"foundation.mechanical.translational.translational\"}],\"Top\":[]}"
  Force Bumpstop : fl_lib/Mechanical/Mechanical Sensors/Ideal Force Sensor
  Force Damper : fl_lib/Mechanical/Mechanical Sensors/Ideal Force Sensor
  Motion Damper : fl_lib/Mechanical/Mechanical Sensors/Ideal Translational Motion Sensor  reference=foundation.enum.MeasurementReference.difference  acceleration_port=false  velocity_port=true  position_port=true  offset=dam_x0 m
  PS-Simulink Converter : nesl_utility/PS-Simulink Converter  PhysicalDomain=network_engine_domain  SubClassName=ps_output  LeftPortType=input  RightPortType=output  PseudoPeriodic=off  Frequencies=[]  VectorFormat=1-D array  Unit=N  AffineConversion=off
  PS-Simulink Converter1 : nesl_utility/PS-Simulink Converter  PhysicalDomain=network_engine_domain  SubClassName=ps_output  LeftPortType=input  RightPortType=output  PseudoPeriodic=off  Frequencies=[]  VectorFormat=1-D array  Unit=N  AffineConversion=off
  PS-Simulink Converter2 : nesl_utility/PS-Simulink Converter  PhysicalDomain=network_engine_domain  SubClassName=ps_output  LeftPortType=input  RightPortType=output  PseudoPeriodic=off  Frequencies=[]  VectorFormat=1-D array  Unit=m/s  AffineConversion=off
  PS-Simulink Converter3 : nesl_utility/PS-Simulink Converter  PhysicalDomain=network_engine_domain  SubClassName=ps_output  LeftPortType=input  RightPortType=output  PseudoPeriodic=off  Frequencies=[]  VectorFormat=1-D array  Unit=m  AffineConversion=off
  Terminator : Terminator
  R : PMIOPort  Side=Left
  C : PMIOPort  Port=2  Side=Right
  Out Bus Element : Outport  VectorParamsAs1DForOutWhenUnconnected=off  PortName=meas  Element=FDamper
  Out Bus Element1 : Outport  VectorParamsAs1DForOutWhenUnconnected=off  PortName=meas  Element=FBumpstop
  Out Bus Element2 : Outport  VectorParamsAs1DForOutWhenUnconnected=off  PortName=meas  Element=xDamper
  Out Bus Element3 : Outport  VectorParamsAs1DForOutWhenUnconnected=off  PortName=meas  Element=vDamper
  wires:
  Ctrl/1 -> Terminator/1
  PS-Simulink Converter/1 -> Out Bus Element/1
  PS-Simulink Converter2/1 -> Out Bus Element3/1
  PS-Simulink Converter3/1 -> Out Bus Element2/1
  PS-Simulink Converter1/1 -> Out Bus Element1/1
  connections:
  Motion Damper/RConn1 -- Force Bumpstop/LConn1 -- C/RConn1 -- Force Damper/LConn1
  PS-Simulink Converter2/LConn1 -- Motion Damper/RConn2
  PS-Simulink Converter1/LConn1 -- Force Bumpstop/RConn2
  PS-Simulink Converter3/LConn1 -- Motion Damper/RConn3
  PS-Simulink Converter/LConn1 -- Force Damper/RConn2
  Force Bumpstop/RConn1 -- Bumpstop/RConn1
  Damper/RConn1 -- Force Damper/RConn1
  Motion Damper/LConn1 -- R/RConn1 -- Bumpstop/LConn1 -- Damper/LConn1

== system sm_car/Vehicle/Vehicle/Chassis/Damper/Decoupled/Damper A1 Heave/Variable ==
  note: Sensing
  Ctrl : Inport
  Bumpstop : fl_lib/Mechanical/Translational Elements/Translational Hard Stop  upper_bnd=bs_lim_upper m  lower_bnd=bs_lim_lower m  model=1  stiff_up=bs_k_upper N/m  stiff_low=bs_k_lower N/m  D_up=bs_b_upper N/(m/s)  D_low=bs_b_lower N/(m/s)  transition=bs_region m  coeff_rest=0.7  v_tol=0.001 m/s  f_tol=0.001 N  v_specify=off  v_priority=None  v=0 m/s  v_nominal_specify=off  v_nominal_value=1  v_nominal_unit=m/s  f_specify=off  f_priority=None  f=0 N  f_nominal_specify=off  f_nominal_value=1  f_nominal_unit=N  x_specify=off  x_priority=High  x=0 m  x_nominal_specify=off  x_nominal_value=1  x_nominal_unit=m  M_specify=off  M_priority=None  M=0
  Damper : sdl_lib/Couplings & Drives/Springs & Dampers/Variable Translational Damper  Bmin=0 N*s/m
      settings: InternalSimscapePortConfiguration="{\"Bottom\":[],\"Left\":[{\"id\":\"B\",\"label\":\"B\",\"type\":\"input\"},{\"id\":\"R\",\"label\":\"R\",\"type\":\"foundation.mechanical.translational.translational\"}],\"Right\":[{\"id\":\"C\",\"label\":\"C\",\"type\":\"foundation.mechanical.translational.translational\"}],\"Top\":[]}"
  Force Bumpstop : fl_lib/Mechanical/Mechanical Sensors/Ideal Force Sensor
  Force Damper : fl_lib/Mechanical/Mechanical Sensors/Ideal Force Sensor
  Motion Damper : fl_lib/Mechanical/Mechanical Sensors/Ideal Translational Motion Sensor  reference=foundation.enum.MeasurementReference.difference  acceleration_port=false  velocity_port=true  position_port=true  offset=dam_x0 m
  PS-Simulink Converter : nesl_utility/PS-Simulink Converter  PhysicalDomain=network_engine_domain  SubClassName=ps_output  LeftPortType=input  RightPortType=output  PseudoPeriodic=off  Frequencies=[]  VectorFormat=1-D array  Unit=N  AffineConversion=off
  PS-Simulink Converter1 : nesl_utility/PS-Simulink Converter  PhysicalDomain=network_engine_domain  SubClassName=ps_output  LeftPortType=input  RightPortType=output  PseudoPeriodic=off  Frequencies=[]  VectorFormat=1-D array  Unit=N  AffineConversion=off
  PS-Simulink Converter2 : nesl_utility/PS-Simulink Converter  PhysicalDomain=network_engine_domain  SubClassName=ps_output  LeftPortType=input  RightPortType=output  PseudoPeriodic=off  Frequencies=[]  VectorFormat=1-D array  Unit=m/s  AffineConversion=off
  PS-Simulink Converter3 : nesl_utility/PS-Simulink Converter  PhysicalDomain=network_engine_domain  SubClassName=ps_output  LeftPortType=input  RightPortType=output  PseudoPeriodic=off  Frequencies=[]  VectorFormat=1-D array  Unit=m  AffineConversion=off
  Simulink-PS Converter : nesl_utility/Simulink-PS Converter  PhysicalDomain=network_engine_domain  SubClassName=ps_input  LeftPortType=input  RightPortType=output  PseudoPeriodic=off  Frequencies=[]  NoiseDistribution=none  NoiseParameters=[]  Unit=N*s/m  AffineConversion=off  FilteringAndDerivatives=provide  SimscapeFilterOrder=1  InputFilterTimeConstant=0.001  UdotUserProvided=0
  R : PMIOPort  Side=Left
  C : PMIOPort  Port=2  Side=Right
  Out Bus Element : Outport  VectorParamsAs1DForOutWhenUnconnected=off  PortName=meas  Element=FDamper
  Out Bus Element1 : Outport  VectorParamsAs1DForOutWhenUnconnected=off  PortName=meas  Element=FBumpstop
  Out Bus Element2 : Outport  VectorParamsAs1DForOutWhenUnconnected=off  PortName=meas  Element=xDamper
  Out Bus Element3 : Outport  VectorParamsAs1DForOutWhenUnconnected=off  PortName=meas  Element=vDamper
  wires:
  PS-Simulink Converter1/1 -> Out Bus Element1/1
  PS-Simulink Converter3/1 -> Out Bus Element2/1
  PS-Simulink Converter2/1 -> Out Bus Element3/1
  PS-Simulink Converter/1 -> Out Bus Element/1
  Ctrl/1 -> Simulink-PS Converter/1
  connections:
  Simulink-PS Converter/RConn1 -- Damper/LConn1
  R/RConn1 -- Motion Damper/LConn1 -- Damper/LConn2 -- Bumpstop/LConn1
  Force Damper/RConn1 -- Damper/RConn1
  Force Bumpstop/RConn1 -- Bumpstop/RConn1
  PS-Simulink Converter/LConn1 -- Force Damper/RConn2
  PS-Simulink Converter3/LConn1 -- Motion Damper/RConn3
  PS-Simulink Converter1/LConn1 -- Force Bumpstop/RConn2
  PS-Simulink Converter2/LConn1 -- Motion Damper/RConn2
  Force Damper/LConn1 -- C/RConn1 -- Force Bumpstop/LConn1 -- Motion Damper/RConn1
